simulink model "BMS4Cell"  (R2026a)
settings: Solver=daessc  StopTime=P.StopTime  MaxStep=10  RelTol=1e-4
InitFcn:
  | addpath(fullfile(fileparts(get_param(bdroot, 'FileName')), '..', 'src')); if ~exist('P','var') || ~exist('C','var'), [P, C] = params_4cell('cell'); end
undefined symbols (not defined in the file): C, P
libraries: fl_lib x39, nesl_utility x28, batteryecm_lib x4, ee_lib x4
settings Model: Creator=highdreameater  LastModifiedBy=highdreameater
settings DebuggingCC: AlgebraicLoopMsg=error

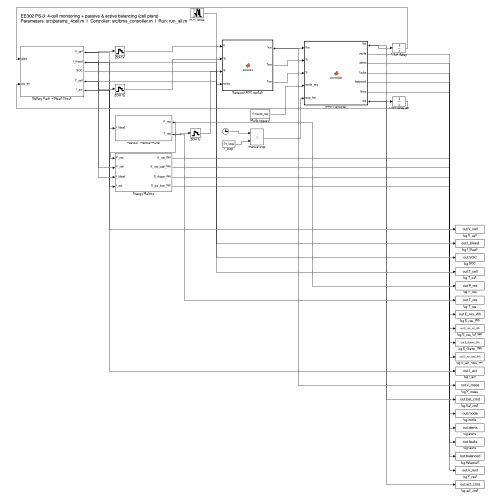
[thumbnail: Simulink's stored preview of the top-level diagram]
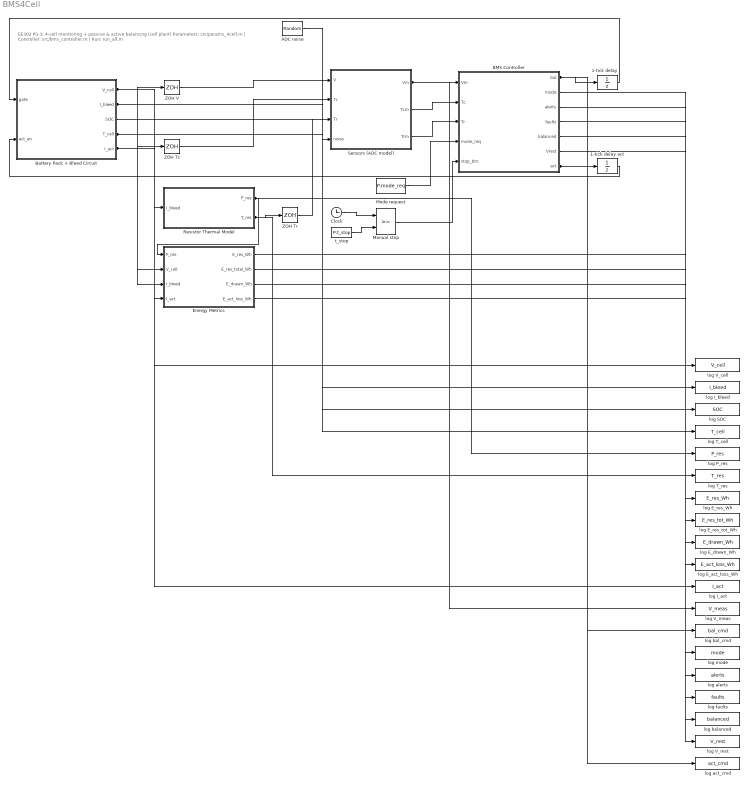
== system BMS4Cell ==
  note: EE302 PS-3: 4-cell monitoring + passive & active balancing (cell plant)
      | Parameters: src/params_4cell.m  |  Controller: src/bms_controller.m  |  Run: run_all.m
  1-tick delay : UnitDelay  InitialCondition=zeros(4,1)  SampleTime=C.Ts
  1-tick delay act : UnitDelay  InitialCondition=zeros(3,1)  SampleTime=C.Ts
  ADC noise : RandomNumber  Mean=zeros(4,1)  Variance=P.noise_V^2*ones(4,1)  Seed=P.seed  SampleTime=C.Ts
  BMS Controller : MATLAB Function  TreatAsAtomicUnit=on
  Battery Pack + Bleed Circuit : Subsystem
  Clock : Clock
  Energy Metrics : Subsystem
  Manual stop : RelationalOperator  OutDataTypeStr=boolean  RndMeth=Simplest  InputSameDT=off
  Mode request : Constant  Value=P.mode_req
  Resistor Thermal Model : Subsystem
  Sensors (ADC model) : MATLAB Function  TreatAsAtomicUnit=on
  ZOH Tc : ZeroOrderHold  SampleTime=C.Ts
  ZOH Tr : ZeroOrderHold  SampleTime=C.Ts
  ZOH V : ZeroOrderHold  SampleTime=C.Ts
  log E_act_loss_Wh : ToWorkspace  VariableName=E_act_loss_Wh  SaveFormat=Timeseries  SampleTime=P.log_dt
  log E_drawn_Wh : ToWorkspace  VariableName=E_drawn_Wh  SaveFormat=Timeseries  SampleTime=P.log_dt
  log E_res_Wh : ToWorkspace  VariableName=E_res_Wh  SaveFormat=Timeseries  SampleTime=P.log_dt
  log E_res_tot_Wh : ToWorkspace  VariableName=E_res_tot_Wh  SaveFormat=Timeseries  SampleTime=P.log_dt
  log I_act : ToWorkspace  VariableName=I_act  SaveFormat=Timeseries  SampleTime=P.log_dt
  log I_bleed : ToWorkspace  VariableName=I_bleed  SaveFormat=Timeseries  SampleTime=P.log_dt
  log P_res : ToWorkspace  VariableName=P_res  SaveFormat=Timeseries  SampleTime=P.log_dt
  log SOC : ToWorkspace  VariableName=SOC  SaveFormat=Timeseries  SampleTime=P.log_dt
  log T_cell : ToWorkspace  VariableName=T_cell  SaveFormat=Timeseries  SampleTime=P.log_dt
  log T_res : ToWorkspace  VariableName=T_res  SaveFormat=Timeseries  SampleTime=P.log_dt
  log V_cell : ToWorkspace  VariableName=V_cell  SaveFormat=Timeseries  SampleTime=P.log_dt
  log V_meas : ToWorkspace  VariableName=V_meas  SaveFormat=Timeseries  SampleTime=C.Ts
  log V_rest : ToWorkspace  VariableName=V_rest  SaveFormat=Timeseries  SampleTime=C.Ts
  log act_cmd : ToWorkspace  VariableName=act_cmd  SaveFormat=Timeseries  SampleTime=C.Ts
  log alerts : ToWorkspace  VariableName=alerts  SaveFormat=Timeseries  SampleTime=C.Ts
  log bal_cmd : ToWorkspace  VariableName=bal_cmd  SaveFormat=Timeseries  SampleTime=C.Ts
  log balanced : ToWorkspace  VariableName=balanced  SaveFormat=Timeseries  SampleTime=C.Ts
  log faults : ToWorkspace  VariableName=faults  SaveFormat=Timeseries  SampleTime=C.Ts
  log mode : ToWorkspace  VariableName=mode  SaveFormat=Timeseries  SampleTime=C.Ts
  t_stop : Constant  Value=P.t_stop
  wires:
  Battery Pack + Bleed Circuit/1(V_cell) -> ZOH V/1, Energy Metrics/2(V_cell), log V_cell/1
  Battery Pack + Bleed Circuit/4(T_cell) -> ZOH Tc/1, log T_cell/1
  Battery Pack + Bleed Circuit/2(I_bleed) -> Resistor Thermal Model/1(I_bleed), Energy Metrics/3(I_bleed), log I_bleed/1
  Resistor Thermal Model/2(T_res) -> ZOH Tr/1, log T_res/1
  Resistor Thermal Model/1(P_res) -> Energy Metrics/1(P_res), log P_res/1
  ZOH V/1 -> Sensors (ADC model)/1(V)
  ZOH Tc/1 -> Sensors (ADC model)/2(Tc)
  ZOH Tr/1 -> Sensors (ADC model)/3(Tr)
  ADC noise/1 -> Sensors (ADC model)/4(noise)
  Sensors (ADC model)/1(Vm) -> BMS Controller/1(Vm), log V_meas/1
  Sensors (ADC model)/2(Tcm) -> BMS Controller/2(Tc)
  Sensors (ADC model)/3(Trm) -> BMS Controller/3(Tr)
  Mode request/1 -> BMS Controller/4(mode_req)
  Clock/1 -> Manual stop/1
  t_stop/1 -> Manual stop/2
  Manual stop/1 -> BMS Controller/5(stop_btn)
  BMS Controller/1(bal) -> 1-tick delay/1, log bal_cmd/1
  1-tick delay/1 -> Battery Pack + Bleed Circuit/1(gate)
  BMS Controller/7(act) -> 1-tick delay act/1, log act_cmd/1
  1-tick delay act/1 -> Battery Pack + Bleed Circuit/2(act_en)
  Battery Pack + Bleed Circuit/5(I_act) -> Energy Metrics/4(I_act), log I_act/1
  Battery Pack + Bleed Circuit/3(SOC) -> log SOC/1
  Energy Metrics/1(E_res_Wh) -> log E_res_Wh/1
  Energy Metrics/2(E_res_total_Wh) -> log E_res_tot_Wh/1
  Energy Metrics/3(E_drawn_Wh) -> log E_drawn_Wh/1
  Energy Metrics/4(E_act_loss_Wh) -> log E_act_loss_Wh/1
  BMS Controller/2(mode) -> log mode/1
  BMS Controller/3(alerts) -> log alerts/1
  BMS Controller/4(faults) -> log faults/1
  BMS Controller/5(balanced) -> log balanced/1
  BMS Controller/6(Vrest) -> log V_rest/1

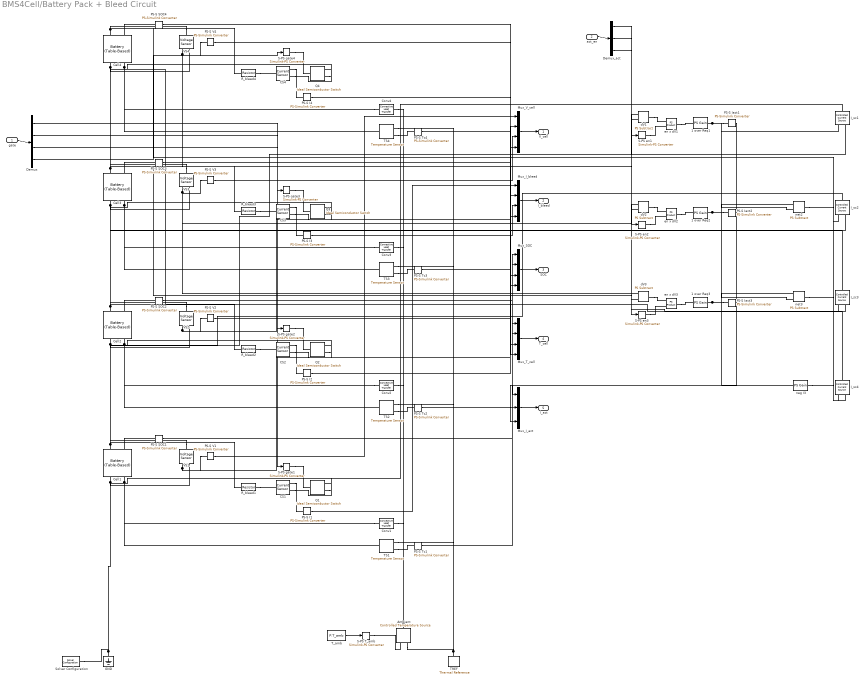
== system BMS4Cell/Battery Pack + Bleed Circuit ==
  gate : Inport
  act_en : Inport  Port=2
  1 over Req1 : fl_lib/Physical Signals/Functions/PS Gain  gain=1/P.R_eq 1/Ohm
  1 over Req2 : fl_lib/Physical Signals/Functions/PS Gain  gain=1/P.R_eq 1/Ohm
  1 over Req3 : fl_lib/Physical Signals/Functions/PS Gain  gain=1/P.R_eq 1/Ohm
  Ambient : fl_lib/Thermal/Thermal Sources/Controlled Temperature Source
  CS{1..4} (4 alike) : fl_lib/Electrical/Electrical Sensors/Current Sensor
  Cell1 : batteryecm_lib/Battery (Table-Based)  SOC_vec=P.SOC_vec  T_dependence=simscape.enum.tablebattery.temperature_dependence.yes  prm_dir=simscape.enum.tablebattery.prm_dir.noCurrentDirectionality  T_vec=P.T_vec K  V0_mat=P.V0_mat V  V0_vec=[3.5057, 3.566, 3.6337, 3.7127, 3.9259, 4.0777, 4.1928] V  V_range=[0, inf] V  R0_mat=P.R0_mat Ohm  R0_vec=[.0085, .0085, .0087, .0082, .0083, .0085, .0085] Ohm  R0_dis_mat=[.0117, .0085, .009; .011, .0085, .009; .0114, .0087, .0092; .0107, .0082, .0088; .0107, .0083, .0091; .0113, .0085, .0089; .0116, .0085, .0089] Ohm  R0_dis_vec=[.0085, .0085, .0087, .0082, .0083, .0085, .0085] Ohm  R0_ch_mat=[.0117, .0085, .009; .011, .0085, .009; .0114, .0087, .0092; .0107, .0082, .0088; .0107, .0083, .0091; .0113, .0085, .0089; .0116, .0085, .0089] Ohm  R0_ch_vec=[.0085, .0085, .0087, .0082, .0083, .0085, .0085] Ohm  AH=P.AH A*hr  prm_leak=simscape.enum.tablebattery.prm_leak.disabled  Rleak_vec=[8000, 7000, 6000] Ohm  Rleak=7e3 Ohm  extrapolation_option=simscape.enum.extrapolation.nearest  SOC_port=simscape.enum.tablebattery.enable.yes  prm_dyn=simscape.enum.tablebattery.prm_dyn.off  R1_mat=[.0109, .0029, .0013; .0069, .0024, .0012; .0047, .0026, .0013; .0034, .0016, .001; .0033, .0023, .0014; .0033, .0018, .0011; .0028, .0017, .0011] Ohm  R1_vec=[.0029, .0024, .0026, .0016, .0023, .0018, .0017] Ohm  tau1_mat=[20, 36, 39; 31, 45, 39; 109, 105, 61; 36, 29, 26; 59, 77, 67; 40, 33, 29; 25, 39, 33] s  tau1_vec=[36, 45, 105, 29, 77, 33, 39] s  R2_mat=[.0109, .0029, .0013; .0069, .0024, .0012; .0047, .0026, .0013; .0034, .0016, .001; .0033, .0023, .0014; .0033, .0018, .0011; .0028, .0017, .0011] Ohm  R2_vec=[.0029, .0024, .0026, .0016, .0023, .0018, .0017] Ohm  tau2_mat=[20, 36, 39; 31, 45, 39; 109, 105, 61; 36, 29, 26; 59, 77, 67; 40, 33, 29; 25, 39, 33] s  tau2_vec=[36, 45, 105, 29, 77, 33, 39] s  R3_mat=[.0109, .0029, .0013; .0069, .0024, .0012; .0047, .0026, .0013; .0034, .0016, .001; .0033, .0023, .0014; .0033, .0018, .0011; .0028, .0017, .0011] Ohm  R3_vec=[.0029, .0024, .0026, .0016, .0023, .0018, .0017] Ohm  tau3_mat=[20, 36, 39; 31, 45, 39; 109, 105, 61; 36, 29, 26; 59, 77, 67; 40, 33, 29; 25, 39, 33] s  tau3_vec=[36, 45, 105, 29, 77, 33, 39] s  R4_mat=[.0109, .0029, .0013; .0069, .0024, .0012; .0047, .0026, .0013; .0034, .0016, .001; .0033, .0023, .0014; .0033, .0018, .0011; .0028, .0017, .0011] Ohm  R4_vec=[.0029, .0024, .0026, .0016, .0023, .0018, .0017] Ohm  tau4_mat=[20, 36, 39; 31, 45, 39; 109, 105, 61; 36, 29, 26; 59, 77, 67; 40, 33, 29; 25, 39, 33] s  tau4_vec=[36, 45, 105, 29, 77, 33, 39] s  R5_mat=[.0109, .0029, .0013; .0069, .0024, .0012; .0047, .0026, .0013; .0034, .0016, .001; .0033, .0023, .0014; .0033, .0018, .0011; .0028, .0017, .0011] Ohm  R5_vec=[.0029, .0024, .0026, .0016, .0023, .0018, .0017] Ohm  tau5_mat=[20, 36, 39; 31, 45, 39; 109, 105, 61; 36, 29, 26; 59, 77, 67; 40, 33, 29; 25, 39, 33] s  tau5_vec=[36, 45, 105, 29, 77, 33, 39] s  prm_fade=simscape.enum.tablebattery.prm_fade.disabled  N0=100  dV0=0  dR0=0  dAH=0  dRleak=0  dR1=0  dR2=0  dR3=0  dR4=0  dR5=0  N0vec=[0, 100, 200, 300]  Tfadevec=[298.15, 323.15] K  dV0vec=[0, 0, 0, 0]  dR0vec=[0, 0, 0, 0]  dAHvec=[0, 0, 0, 0]  dRleakvec=[0, 0, 0, 0]  dR1vec=[0, 0, 0, 0]  dR2vec=[0, 0, 0, 0]  dR3vec=[0, 0, 0, 0]  dR4vec=[0, 0, 0, 0]  dR5vec=[0, 0, 0, 0]  dV0mat=[0, 0; 0, 0; 0, 0; 0, 0]  dR0mat=[0, 0; 0, 0; 0, 0; 0, 0]  dAHmat=[0, 0; 0, 0; 0, 0; 0, 0]  dRleakmat=[0, 0; 0, 0; 0, 0; 0, 0]  dR1mat=[0, 0; 0, 0; 0, 0; 0, 0]  dR2mat=[0, 0; 0, 0; 0, 0; 0, 0]  dR3mat=[0, 0; 0, 0; 0, 0; 0, 0]  dR4mat=[0, 0; 0, 0; 0, 0; 0, 0]  dR5mat=[0, 0; 0, 0; 0, 0; 0, 0]  prm_age_modeling=simscape.enum.tablebattery.prm_age_modeling.equation  storage_dt_age_vec=[0] d  storage_T_age_vec=[273] K  prm_age_OCV=simscape.enum.tablebattery.prm_age_OCV.OCV  OCV_age=0.9  SOC_age=0.6  prm_age_resistance=simscape.enum.tablebattery.prm_age.disabled  OCV_scaling_age_resistance=2.2134e6  OCV_offset_age_resistance=1.632e6  temp_exp_age_resistance=0.515833569 V  t_exp_age_resistance=0.75  T_age_vec_resistance=[273.15, 298.15, 323.15] K  dt_age_vec_resistance=[0, 90, 180, 270] d  dR0_age_vec=[0, 0, 0]  t_meas_dR0_age=100 d  dR0_age_mat=[0, 0, 0; 0, 0, 0; 0, 0, 0; 0, 0, 0]  prm_age_capacity=simscape.enum.tablebattery.prm_age.disabled  OCV_scaling_age_capacity=1.5097e07  OCV_offset_age_capacity=8.3625e06  temp_exp_age_capacity=0.6011 V  t_exp_age_capacity=0.75  T_age_vec_capacity=[273.15, 298.15, 323.15] K  dt_age_vec_capacity=[0, 90, 180, 270] d  dAH_age_vec=[0, 0, 0]  t_meas_dAH_age=100 d  dAH_age_mat=[0, 0, 0; 0, 0, 0; 0, 0, 0; 0, 0, 0]  thermal_port=simscape.enum.thermaleffects.model  temperature=298.15 K  thermal_mass=P.Cth_cell J/K  i_specify=off  i_priority=None  i=0 A  i_nominal_specify=off  i_nominal_value=1  i_nominal_unit=A  v_specify=off  v_priority=None  v=0 V  v_nominal_specify=off  v_nominal_value=1  v_nominal_unit=V  stateOfCharge_specify=on  stateOfCharge_priority=High  stateOfCharge=P.SOC0(1)  stateOfCharge_nominal_specify=off  stateOfCharge_nominal_value=1  stateOfCharge_nominal_unit=1  num_cycles_specify=off  num_cycles_priority=High  num_cycles=0  num_cycles_nominal_specify=off  num_cycles_nominal_value=1  num_cycles_nominal_unit=1  cell_temperature_specify=on  cell_temperature_priority=High  cell_temperature=P.T_amb + 273.15 K  cell_temperature_nominal_specify=off  cell_temperature_nominal_value=1  cell_temperature_nominal_unit=K
  Cell2 : batteryecm_lib/Battery (Table-Based)  SOC_vec=P.SOC_vec  T_dependence=simscape.enum.tablebattery.temperature_dependence.yes  prm_dir=simscape.enum.tablebattery.prm_dir.noCurrentDirectionality  T_vec=P.T_vec K  V0_mat=P.V0_mat V  V0_vec=[3.5057, 3.566, 3.6337, 3.7127, 3.9259, 4.0777, 4.1928] V  V_range=[0, inf] V  R0_mat=P.R0_mat Ohm  R0_vec=[.0085, .0085, .0087, .0082, .0083, .0085, .0085] Ohm  R0_dis_mat=[.0117, .0085, .009; .011, .0085, .009; .0114, .0087, .0092; .0107, .0082, .0088; .0107, .0083, .0091; .0113, .0085, .0089; .0116, .0085, .0089] Ohm  R0_dis_vec=[.0085, .0085, .0087, .0082, .0083, .0085, .0085] Ohm  R0_ch_mat=[.0117, .0085, .009; .011, .0085, .009; .0114, .0087, .0092; .0107, .0082, .0088; .0107, .0083, .0091; .0113, .0085, .0089; .0116, .0085, .0089] Ohm  R0_ch_vec=[.0085, .0085, .0087, .0082, .0083, .0085, .0085] Ohm  AH=P.AH A*hr  prm_leak=simscape.enum.tablebattery.prm_leak.disabled  Rleak_vec=[8000, 7000, 6000] Ohm  Rleak=7e3 Ohm  extrapolation_option=simscape.enum.extrapolation.nearest  SOC_port=simscape.enum.tablebattery.enable.yes  prm_dyn=simscape.enum.tablebattery.prm_dyn.off  R1_mat=[.0109, .0029, .0013; .0069, .0024, .0012; .0047, .0026, .0013; .0034, .0016, .001; .0033, .0023, .0014; .0033, .0018, .0011; .0028, .0017, .0011] Ohm  R1_vec=[.0029, .0024, .0026, .0016, .0023, .0018, .0017] Ohm  tau1_mat=[20, 36, 39; 31, 45, 39; 109, 105, 61; 36, 29, 26; 59, 77, 67; 40, 33, 29; 25, 39, 33] s  tau1_vec=[36, 45, 105, 29, 77, 33, 39] s  R2_mat=[.0109, .0029, .0013; .0069, .0024, .0012; .0047, .0026, .0013; .0034, .0016, .001; .0033, .0023, .0014; .0033, .0018, .0011; .0028, .0017, .0011] Ohm  R2_vec=[.0029, .0024, .0026, .0016, .0023, .0018, .0017] Ohm  tau2_mat=[20, 36, 39; 31, 45, 39; 109, 105, 61; 36, 29, 26; 59, 77, 67; 40, 33, 29; 25, 39, 33] s  tau2_vec=[36, 45, 105, 29, 77, 33, 39] s  R3_mat=[.0109, .0029, .0013; .0069, .0024, .0012; .0047, .0026, .0013; .0034, .0016, .001; .0033, .0023, .0014; .0033, .0018, .0011; .0028, .0017, .0011] Ohm  R3_vec=[.0029, .0024, .0026, .0016, .0023, .0018, .0017] Ohm  tau3_mat=[20, 36, 39; 31, 45, 39; 109, 105, 61; 36, 29, 26; 59, 77, 67; 40, 33, 29; 25, 39, 33] s  tau3_vec=[36, 45, 105, 29, 77, 33, 39] s  R4_mat=[.0109, .0029, .0013; .0069, .0024, .0012; .0047, .0026, .0013; .0034, .0016, .001; .0033, .0023, .0014; .0033, .0018, .0011; .0028, .0017, .0011] Ohm  R4_vec=[.0029, .0024, .0026, .0016, .0023, .0018, .0017] Ohm  tau4_mat=[20, 36, 39; 31, 45, 39; 109, 105, 61; 36, 29, 26; 59, 77, 67; 40, 33, 29; 25, 39, 33] s  tau4_vec=[36, 45, 105, 29, 77, 33, 39] s  R5_mat=[.0109, .0029, .0013; .0069, .0024, .0012; .0047, .0026, .0013; .0034, .0016, .001; .0033, .0023, .0014; .0033, .0018, .0011; .0028, .0017, .0011] Ohm  R5_vec=[.0029, .0024, .0026, .0016, .0023, .0018, .0017] Ohm  tau5_mat=[20, 36, 39; 31, 45, 39; 109, 105, 61; 36, 29, 26; 59, 77, 67; 40, 33, 29; 25, 39, 33] s  tau5_vec=[36, 45, 105, 29, 77, 33, 39] s  prm_fade=simscape.enum.tablebattery.prm_fade.disabled  N0=100  dV0=0  dR0=0  dAH=0  dRleak=0  dR1=0  dR2=0  dR3=0  dR4=0  dR5=0  N0vec=[0, 100, 200, 300]  Tfadevec=[298.15, 323.15] K  dV0vec=[0, 0, 0, 0]  dR0vec=[0, 0, 0, 0]  dAHvec=[0, 0, 0, 0]  dRleakvec=[0, 0, 0, 0]  dR1vec=[0, 0, 0, 0]  dR2vec=[0, 0, 0, 0]  dR3vec=[0, 0, 0, 0]  dR4vec=[0, 0, 0, 0]  dR5vec=[0, 0, 0, 0]  dV0mat=[0, 0; 0, 0; 0, 0; 0, 0]  dR0mat=[0, 0; 0, 0; 0, 0; 0, 0]  dAHmat=[0, 0; 0, 0; 0, 0; 0, 0]  dRleakmat=[0, 0; 0, 0; 0, 0; 0, 0]  dR1mat=[0, 0; 0, 0; 0, 0; 0, 0]  dR2mat=[0, 0; 0, 0; 0, 0; 0, 0]  dR3mat=[0, 0; 0, 0; 0, 0; 0, 0]  dR4mat=[0, 0; 0, 0; 0, 0; 0, 0]  dR5mat=[0, 0; 0, 0; 0, 0; 0, 0]  prm_age_modeling=simscape.enum.tablebattery.prm_age_modeling.equation  storage_dt_age_vec=[0] d  storage_T_age_vec=[273] K  prm_age_OCV=simscape.enum.tablebattery.prm_age_OCV.OCV  OCV_age=0.9  SOC_age=0.6  prm_age_resistance=simscape.enum.tablebattery.prm_age.disabled  OCV_scaling_age_resistance=2.2134e6  OCV_offset_age_resistance=1.632e6  temp_exp_age_resistance=0.515833569 V  t_exp_age_resistance=0.75  T_age_vec_resistance=[273.15, 298.15, 323.15] K  dt_age_vec_resistance=[0, 90, 180, 270] d  dR0_age_vec=[0, 0, 0]  t_meas_dR0_age=100 d  dR0_age_mat=[0, 0, 0; 0, 0, 0; 0, 0, 0; 0, 0, 0]  prm_age_capacity=simscape.enum.tablebattery.prm_age.disabled  OCV_scaling_age_capacity=1.5097e07  OCV_offset_age_capacity=8.3625e06  temp_exp_age_capacity=0.6011 V  t_exp_age_capacity=0.75  T_age_vec_capacity=[273.15, 298.15, 323.15] K  dt_age_vec_capacity=[0, 90, 180, 270] d  dAH_age_vec=[0, 0, 0]  t_meas_dAH_age=100 d  dAH_age_mat=[0, 0, 0; 0, 0, 0; 0, 0, 0; 0, 0, 0]  thermal_port=simscape.enum.thermaleffects.model  temperature=298.15 K  thermal_mass=P.Cth_cell J/K  i_specify=off  i_priority=None  i=0 A  i_nominal_specify=off  i_nominal_value=1  i_nominal_unit=A  v_specify=off  v_priority=None  v=0 V  v_nominal_specify=off  v_nominal_value=1  v_nominal_unit=V  stateOfCharge_specify=on  stateOfCharge_priority=High  stateOfCharge=P.SOC0(2)  stateOfCharge_nominal_specify=off  stateOfCharge_nominal_value=1  stateOfCharge_nominal_unit=1  num_cycles_specify=off  num_cycles_priority=High  num_cycles=0  num_cycles_nominal_specify=off  num_cycles_nominal_value=1  num_cycles_nominal_unit=1  cell_temperature_specify=on  cell_temperature_priority=High  cell_temperature=P.T_amb + 273.15 K  cell_temperature_nominal_specify=off  cell_temperature_nominal_value=1  cell_temperature_nominal_unit=K
  Cell3 : batteryecm_lib/Battery (Table-Based)  SOC_vec=P.SOC_vec  T_dependence=simscape.enum.tablebattery.temperature_dependence.yes  prm_dir=simscape.enum.tablebattery.prm_dir.noCurrentDirectionality  T_vec=P.T_vec K  V0_mat=P.V0_mat V  V0_vec=[3.5057, 3.566, 3.6337, 3.7127, 3.9259, 4.0777, 4.1928] V  V_range=[0, inf] V  R0_mat=P.R0_mat Ohm  R0_vec=[.0085, .0085, .0087, .0082, .0083, .0085, .0085] Ohm  R0_dis_mat=[.0117, .0085, .009; .011, .0085, .009; .0114, .0087, .0092; .0107, .0082, .0088; .0107, .0083, .0091; .0113, .0085, .0089; .0116, .0085, .0089] Ohm  R0_dis_vec=[.0085, .0085, .0087, .0082, .0083, .0085, .0085] Ohm  R0_ch_mat=[.0117, .0085, .009; .011, .0085, .009; .0114, .0087, .0092; .0107, .0082, .0088; .0107, .0083, .0091; .0113, .0085, .0089; .0116, .0085, .0089] Ohm  R0_ch_vec=[.0085, .0085, .0087, .0082, .0083, .0085, .0085] Ohm  AH=P.AH A*hr  prm_leak=simscape.enum.tablebattery.prm_leak.disabled  Rleak_vec=[8000, 7000, 6000] Ohm  Rleak=7e3 Ohm  extrapolation_option=simscape.enum.extrapolation.nearest  SOC_port=simscape.enum.tablebattery.enable.yes  prm_dyn=simscape.enum.tablebattery.prm_dyn.off  R1_mat=[.0109, .0029, .0013; .0069, .0024, .0012; .0047, .0026, .0013; .0034, .0016, .001; .0033, .0023, .0014; .0033, .0018, .0011; .0028, .0017, .0011] Ohm  R1_vec=[.0029, .0024, .0026, .0016, .0023, .0018, .0017] Ohm  tau1_mat=[20, 36, 39; 31, 45, 39; 109, 105, 61; 36, 29, 26; 59, 77, 67; 40, 33, 29; 25, 39, 33] s  tau1_vec=[36, 45, 105, 29, 77, 33, 39] s  R2_mat=[.0109, .0029, .0013; .0069, .0024, .0012; .0047, .0026, .0013; .0034, .0016, .001; .0033, .0023, .0014; .0033, .0018, .0011; .0028, .0017, .0011] Ohm  R2_vec=[.0029, .0024, .0026, .0016, .0023, .0018, .0017] Ohm  tau2_mat=[20, 36, 39; 31, 45, 39; 109, 105, 61; 36, 29, 26; 59, 77, 67; 40, 33, 29; 25, 39, 33] s  tau2_vec=[36, 45, 105, 29, 77, 33, 39] s  R3_mat=[.0109, .0029, .0013; .0069, .0024, .0012; .0047, .0026, .0013; .0034, .0016, .001; .0033, .0023, .0014; .0033, .0018, .0011; .0028, .0017, .0011] Ohm  R3_vec=[.0029, .0024, .0026, .0016, .0023, .0018, .0017] Ohm  tau3_mat=[20, 36, 39; 31, 45, 39; 109, 105, 61; 36, 29, 26; 59, 77, 67; 40, 33, 29; 25, 39, 33] s  tau3_vec=[36, 45, 105, 29, 77, 33, 39] s  R4_mat=[.0109, .0029, .0013; .0069, .0024, .0012; .0047, .0026, .0013; .0034, .0016, .001; .0033, .0023, .0014; .0033, .0018, .0011; .0028, .0017, .0011] Ohm  R4_vec=[.0029, .0024, .0026, .0016, .0023, .0018, .0017] Ohm  tau4_mat=[20, 36, 39; 31, 45, 39; 109, 105, 61; 36, 29, 26; 59, 77, 67; 40, 33, 29; 25, 39, 33] s  tau4_vec=[36, 45, 105, 29, 77, 33, 39] s  R5_mat=[.0109, .0029, .0013; .0069, .0024, .0012; .0047, .0026, .0013; .0034, .0016, .001; .0033, .0023, .0014; .0033, .0018, .0011; .0028, .0017, .0011] Ohm  R5_vec=[.0029, .0024, .0026, .0016, .0023, .0018, .0017] Ohm  tau5_mat=[20, 36, 39; 31, 45, 39; 109, 105, 61; 36, 29, 26; 59, 77, 67; 40, 33, 29; 25, 39, 33] s  tau5_vec=[36, 45, 105, 29, 77, 33, 39] s  prm_fade=simscape.enum.tablebattery.prm_fade.disabled  N0=100  dV0=0  dR0=0  dAH=0  dRleak=0  dR1=0  dR2=0  dR3=0  dR4=0  dR5=0  N0vec=[0, 100, 200, 300]  Tfadevec=[298.15, 323.15] K  dV0vec=[0, 0, 0, 0]  dR0vec=[0, 0, 0, 0]  dAHvec=[0, 0, 0, 0]  dRleakvec=[0, 0, 0, 0]  dR1vec=[0, 0, 0, 0]  dR2vec=[0, 0, 0, 0]  dR3vec=[0, 0, 0, 0]  dR4vec=[0, 0, 0, 0]  dR5vec=[0, 0, 0, 0]  dV0mat=[0, 0; 0, 0; 0, 0; 0, 0]  dR0mat=[0, 0; 0, 0; 0, 0; 0, 0]  dAHmat=[0, 0; 0, 0; 0, 0; 0, 0]  dRleakmat=[0, 0; 0, 0; 0, 0; 0, 0]  dR1mat=[0, 0; 0, 0; 0, 0; 0, 0]  dR2mat=[0, 0; 0, 0; 0, 0; 0, 0]  dR3mat=[0, 0; 0, 0; 0, 0; 0, 0]  dR4mat=[0, 0; 0, 0; 0, 0; 0, 0]  dR5mat=[0, 0; 0, 0; 0, 0; 0, 0]  prm_age_modeling=simscape.enum.tablebattery.prm_age_modeling.equation  storage_dt_age_vec=[0] d  storage_T_age_vec=[273] K  prm_age_OCV=simscape.enum.tablebattery.prm_age_OCV.OCV  OCV_age=0.9  SOC_age=0.6  prm_age_resistance=simscape.enum.tablebattery.prm_age.disabled  OCV_scaling_age_resistance=2.2134e6  OCV_offset_age_resistance=1.632e6  temp_exp_age_resistance=0.515833569 V  t_exp_age_resistance=0.75  T_age_vec_resistance=[273.15, 298.15, 323.15] K  dt_age_vec_resistance=[0, 90, 180, 270] d  dR0_age_vec=[0, 0, 0]  t_meas_dR0_age=100 d  dR0_age_mat=[0, 0, 0; 0, 0, 0; 0, 0, 0; 0, 0, 0]  prm_age_capacity=simscape.enum.tablebattery.prm_age.disabled  OCV_scaling_age_capacity=1.5097e07  OCV_offset_age_capacity=8.3625e06  temp_exp_age_capacity=0.6011 V  t_exp_age_capacity=0.75  T_age_vec_capacity=[273.15, 298.15, 323.15] K  dt_age_vec_capacity=[0, 90, 180, 270] d  dAH_age_vec=[0, 0, 0]  t_meas_dAH_age=100 d  dAH_age_mat=[0, 0, 0; 0, 0, 0; 0, 0, 0; 0, 0, 0]  thermal_port=simscape.enum.thermaleffects.model  temperature=298.15 K  thermal_mass=P.Cth_cell J/K  i_specify=off  i_priority=None  i=0 A  i_nominal_specify=off  i_nominal_value=1  i_nominal_unit=A  v_specify=off  v_priority=None  v=0 V  v_nominal_specify=off  v_nominal_value=1  v_nominal_unit=V  stateOfCharge_specify=on  stateOfCharge_priority=High  stateOfCharge=P.SOC0(3)  stateOfCharge_nominal_specify=off  stateOfCharge_nominal_value=1  stateOfCharge_nominal_unit=1  num_cycles_specify=off  num_cycles_priority=High  num_cycles=0  num_cycles_nominal_specify=off  num_cycles_nominal_value=1  num_cycles_nominal_unit=1  cell_temperature_specify=on  cell_temperature_priority=High  cell_temperature=P.T_amb + 273.15 K  cell_temperature_nominal_specify=off  cell_temperature_nominal_value=1  cell_temperature_nominal_unit=K
  Cell4 : batteryecm_lib/Battery (Table-Based)  SOC_vec=P.SOC_vec  T_dependence=simscape.enum.tablebattery.temperature_dependence.yes  prm_dir=simscape.enum.tablebattery.prm_dir.noCurrentDirectionality  T_vec=P.T_vec K  V0_mat=P.V0_mat V  V0_vec=[3.5057, 3.566, 3.6337, 3.7127, 3.9259, 4.0777, 4.1928] V  V_range=[0, inf] V  R0_mat=P.R0_mat Ohm  R0_vec=[.0085, .0085, .0087, .0082, .0083, .0085, .0085] Ohm  R0_dis_mat=[.0117, .0085, .009; .011, .0085, .009; .0114, .0087, .0092; .0107, .0082, .0088; .0107, .0083, .0091; .0113, .0085, .0089; .0116, .0085, .0089] Ohm  R0_dis_vec=[.0085, .0085, .0087, .0082, .0083, .0085, .0085] Ohm  R0_ch_mat=[.0117, .0085, .009; .011, .0085, .009; .0114, .0087, .0092; .0107, .0082, .0088; .0107, .0083, .0091; .0113, .0085, .0089; .0116, .0085, .0089] Ohm  R0_ch_vec=[.0085, .0085, .0087, .0082, .0083, .0085, .0085] Ohm  AH=P.AH A*hr  prm_leak=simscape.enum.tablebattery.prm_leak.disabled  Rleak_vec=[8000, 7000, 6000] Ohm  Rleak=7e3 Ohm  extrapolation_option=simscape.enum.extrapolation.nearest  SOC_port=simscape.enum.tablebattery.enable.yes  prm_dyn=simscape.enum.tablebattery.prm_dyn.off  R1_mat=[.0109, .0029, .0013; .0069, .0024, .0012; .0047, .0026, .0013; .0034, .0016, .001; .0033, .0023, .0014; .0033, .0018, .0011; .0028, .0017, .0011] Ohm  R1_vec=[.0029, .0024, .0026, .0016, .0023, .0018, .0017] Ohm  tau1_mat=[20, 36, 39; 31, 45, 39; 109, 105, 61; 36, 29, 26; 59, 77, 67; 40, 33, 29; 25, 39, 33] s  tau1_vec=[36, 45, 105, 29, 77, 33, 39] s  R2_mat=[.0109, .0029, .0013; .0069, .0024, .0012; .0047, .0026, .0013; .0034, .0016, .001; .0033, .0023, .0014; .0033, .0018, .0011; .0028, .0017, .0011] Ohm  R2_vec=[.0029, .0024, .0026, .0016, .0023, .0018, .0017] Ohm  tau2_mat=[20, 36, 39; 31, 45, 39; 109, 105, 61; 36, 29, 26; 59, 77, 67; 40, 33, 29; 25, 39, 33] s  tau2_vec=[36, 45, 105, 29, 77, 33, 39] s  R3_mat=[.0109, .0029, .0013; .0069, .0024, .0012; .0047, .0026, .0013; .0034, .0016, .001; .0033, .0023, .0014; .0033, .0018, .0011; .0028, .0017, .0011] Ohm  R3_vec=[.0029, .0024, .0026, .0016, .0023, .0018, .0017] Ohm  tau3_mat=[20, 36, 39; 31, 45, 39; 109, 105, 61; 36, 29, 26; 59, 77, 67; 40, 33, 29; 25, 39, 33] s  tau3_vec=[36, 45, 105, 29, 77, 33, 39] s  R4_mat=[.0109, .0029, .0013; .0069, .0024, .0012; .0047, .0026, .0013; .0034, .0016, .001; .0033, .0023, .0014; .0033, .0018, .0011; .0028, .0017, .0011] Ohm  R4_vec=[.0029, .0024, .0026, .0016, .0023, .0018, .0017] Ohm  tau4_mat=[20, 36, 39; 31, 45, 39; 109, 105, 61; 36, 29, 26; 59, 77, 67; 40, 33, 29; 25, 39, 33] s  tau4_vec=[36, 45, 105, 29, 77, 33, 39] s  R5_mat=[.0109, .0029, .0013; .0069, .0024, .0012; .0047, .0026, .0013; .0034, .0016, .001; .0033, .0023, .0014; .0033, .0018, .0011; .0028, .0017, .0011] Ohm  R5_vec=[.0029, .0024, .0026, .0016, .0023, .0018, .0017] Ohm  tau5_mat=[20, 36, 39; 31, 45, 39; 109, 105, 61; 36, 29, 26; 59, 77, 67; 40, 33, 29; 25, 39, 33] s  tau5_vec=[36, 45, 105, 29, 77, 33, 39] s  prm_fade=simscape.enum.tablebattery.prm_fade.disabled  N0=100  dV0=0  dR0=0  dAH=0  dRleak=0  dR1=0  dR2=0  dR3=0  dR4=0  dR5=0  N0vec=[0, 100, 200, 300]  Tfadevec=[298.15, 323.15] K  dV0vec=[0, 0, 0, 0]  dR0vec=[0, 0, 0, 0]  dAHvec=[0, 0, 0, 0]  dRleakvec=[0, 0, 0, 0]  dR1vec=[0, 0, 0, 0]  dR2vec=[0, 0, 0, 0]  dR3vec=[0, 0, 0, 0]  dR4vec=[0, 0, 0, 0]  dR5vec=[0, 0, 0, 0]  dV0mat=[0, 0; 0, 0; 0, 0; 0, 0]  dR0mat=[0, 0; 0, 0; 0, 0; 0, 0]  dAHmat=[0, 0; 0, 0; 0, 0; 0, 0]  dRleakmat=[0, 0; 0, 0; 0, 0; 0, 0]  dR1mat=[0, 0; 0, 0; 0, 0; 0, 0]  dR2mat=[0, 0; 0, 0; 0, 0; 0, 0]  dR3mat=[0, 0; 0, 0; 0, 0; 0, 0]  dR4mat=[0, 0; 0, 0; 0, 0; 0, 0]  dR5mat=[0, 0; 0, 0; 0, 0; 0, 0]  prm_age_modeling=simscape.enum.tablebattery.prm_age_modeling.equation  storage_dt_age_vec=[0] d  storage_T_age_vec=[273] K  prm_age_OCV=simscape.enum.tablebattery.prm_age_OCV.OCV  OCV_age=0.9  SOC_age=0.6  prm_age_resistance=simscape.enum.tablebattery.prm_age.disabled  OCV_scaling_age_resistance=2.2134e6  OCV_offset_age_resistance=1.632e6  temp_exp_age_resistance=0.515833569 V  t_exp_age_resistance=0.75  T_age_vec_resistance=[273.15, 298.15, 323.15] K  dt_age_vec_resistance=[0, 90, 180, 270] d  dR0_age_vec=[0, 0, 0]  t_meas_dR0_age=100 d  dR0_age_mat=[0, 0, 0; 0, 0, 0; 0, 0, 0; 0, 0, 0]  prm_age_capacity=simscape.enum.tablebattery.prm_age.disabled  OCV_scaling_age_capacity=1.5097e07  OCV_offset_age_capacity=8.3625e06  temp_exp_age_capacity=0.6011 V  t_exp_age_capacity=0.75  T_age_vec_capacity=[273.15, 298.15, 323.15] K  dt_age_vec_capacity=[0, 90, 180, 270] d  dAH_age_vec=[0, 0, 0]  t_meas_dAH_age=100 d  dAH_age_mat=[0, 0, 0; 0, 0, 0; 0, 0, 0; 0, 0, 0]  thermal_port=simscape.enum.thermaleffects.model  temperature=298.15 K  thermal_mass=P.Cth_cell J/K  i_specify=off  i_priority=None  i=0 A  i_nominal_specify=off  i_nominal_value=1  i_nominal_unit=A  v_specify=off  v_priority=None  v=0 V  v_nominal_specify=off  v_nominal_value=1  v_nominal_unit=V  stateOfCharge_specify=on  stateOfCharge_priority=High  stateOfCharge=P.SOC0(4)  stateOfCharge_nominal_specify=off  stateOfCharge_nominal_value=1  stateOfCharge_nominal_unit=1  num_cycles_specify=off  num_cycles_priority=High  num_cycles=0  num_cycles_nominal_specify=off  num_cycles_nominal_value=1  num_cycles_nominal_unit=1  cell_temperature_specify=on  cell_temperature_priority=High  cell_temperature=P.T_amb + 273.15 K  cell_temperature_nominal_specify=off  cell_temperature_nominal_value=1  cell_temperature_nominal_unit=K
  Conv{1..4} (4 alike) : fl_lib/Thermal/Thermal Elements/Convective Heat Transfer  thermal_type=foundation.enum.constant_variable.constant  area=P.A_cell m^2  heat_tr_coeff=P.h_conv W/(K*m^2)  min_heat_tr_coeff=1e-3 W/(K*m^2)  T_specify=off  T_priority=None  T=0 K  T_nominal_specify=off  T_nominal_value=1  T_nominal_unit=K  Q_specify=off  Q_priority=None  Q=0 W  Q_nominal_specify=off  Q_nominal_value=1  Q_nominal_unit=W
  Demux : Demux
  Demux_act : Demux  Outputs=3
  GND : fl_lib/Electrical/Electrical Elements/Electrical Reference
  I_sc{1..4} (4 alike) : fl_lib/Electrical/Electrical Sources/Controlled Current Source
  Mux_I_act : Mux  Inputs=3
  Mux_I_bleed : Mux
  Mux_SOC : Mux
  Mux_T_cell : Mux
  Mux_V_cell : Mux
  PS-S I{1..4} (4 alike) : nesl_utility/PS-Simulink Converter  PhysicalDomain=network_engine_domain  SubClassName=ps_output  LeftPortType=input  RightPortType=output  PseudoPeriodic=off  Frequencies=[]  VectorFormat=inherit  Unit=A  AffineConversion=off
  PS-S Iact1 : nesl_utility/PS-Simulink Converter  PhysicalDomain=network_engine_domain  SubClassName=ps_output  LeftPortType=input  RightPortType=output  PseudoPeriodic=off  Frequencies=[]  VectorFormat=inherit  Unit=A  AffineConversion=off
  PS-S Iact2 : nesl_utility/PS-Simulink Converter  PhysicalDomain=network_engine_domain  SubClassName=ps_output  LeftPortType=input  RightPortType=output  PseudoPeriodic=off  Frequencies=[]  VectorFormat=inherit  Unit=A  AffineConversion=off
  PS-S Iact3 : nesl_utility/PS-Simulink Converter  PhysicalDomain=network_engine_domain  SubClassName=ps_output  LeftPortType=input  RightPortType=output  PseudoPeriodic=off  Frequencies=[]  VectorFormat=inherit  Unit=A  AffineConversion=off
  PS-S SOC{1..4} (4 alike) : nesl_utility/PS-Simulink Converter  PhysicalDomain=network_engine_domain  SubClassName=ps_output  LeftPortType=input  RightPortType=output  PseudoPeriodic=off  Frequencies=[]  VectorFormat=inherit  Unit=1  AffineConversion=off
  PS-S Tc{1..4} (4 alike) : nesl_utility/PS-Simulink Converter  PhysicalDomain=network_engine_domain  SubClassName=ps_output  LeftPortType=input  RightPortType=output  PseudoPeriodic=off  Frequencies=[]  VectorFormat=inherit  Unit=degC  AffineConversion=on
  PS-S V{1..4} (4 alike) : nesl_utility/PS-Simulink Converter  PhysicalDomain=network_engine_domain  SubClassName=ps_output  LeftPortType=input  RightPortType=output  PseudoPeriodic=off  Frequencies=[]  VectorFormat=inherit  Unit=V  AffineConversion=off
  Q{1..4} (4 alike) : ee_lib/Semiconductors & Converters/Ideal Semiconductor Switch  port_option=ee.enum.controlport.ps  Ron=P.R_on Ohm  Goff=1e-6 1/Ohm  Vth=0.5 V  diode_param=ee.enum.semiconductors.protectionDiode.external  diode_Vf=0.8 V  diode_Ron=0.001 Ohm  diode_Goff=1e-5 1/Ohm  diode_C=50e-9 F  diode_iRM=-235 A  diode_iF=300 A  diode_idot=-50 A/us  diode_trr_param=ee.enum.converters.diodetrr.trr_factor  diode_trr_factor=3  diode_trr=15 us  diode_Qrr=1500 s*uA
  R_bleed{1..4} (4 alike) : fl_lib/Electrical/Electrical Elements/Resistor  R=P.R_bleed Ohm  i_specify=off  i_priority=None  i=0 A  i_nominal_specify=off  i_nominal_value=1  i_nominal_unit=A  v_specify=off  v_priority=None  v=0 V  v_nominal_specify=off  v_nominal_value=1  v_nominal_unit=V
  S-PS T_amb : nesl_utility/Simulink-PS Converter  PhysicalDomain=network_engine_domain  SubClassName=ps_input  LeftPortType=input  RightPortType=output  PseudoPeriodic=off  Frequencies=[]  NoiseDistribution=none  NoiseParameters=[]  Unit=degC  AffineConversion=on  FilteringAndDerivatives=provide  SimscapeFilterOrder=1  InputFilterTimeConstant=0.001  UdotUserProvided=0
  S-PS en1 : nesl_utility/Simulink-PS Converter  PhysicalDomain=network_engine_domain  SubClassName=ps_input  LeftPortType=input  RightPortType=output  PseudoPeriodic=off  Frequencies=[]  NoiseDistribution=none  NoiseParameters=[]  Unit=1  AffineConversion=off  FilteringAndDerivatives=provide  SimscapeFilterOrder=1  InputFilterTimeConstant=0.001  UdotUserProvided=0
  S-PS en2 : nesl_utility/Simulink-PS Converter  PhysicalDomain=network_engine_domain  SubClassName=ps_input  LeftPortType=input  RightPortType=output  PseudoPeriodic=off  Frequencies=[]  NoiseDistribution=none  NoiseParameters=[]  Unit=1  AffineConversion=off  FilteringAndDerivatives=provide  SimscapeFilterOrder=1  InputFilterTimeConstant=0.001  UdotUserProvided=0
  S-PS en3 : nesl_utility/Simulink-PS Converter  PhysicalDomain=network_engine_domain  SubClassName=ps_input  LeftPortType=input  RightPortType=output  PseudoPeriodic=off  Frequencies=[]  NoiseDistribution=none  NoiseParameters=[]  Unit=1  AffineConversion=off  FilteringAndDerivatives=provide  SimscapeFilterOrder=1  InputFilterTimeConstant=0.001  UdotUserProvided=0
  S-PS gate{1..4} (4 alike) : nesl_utility/Simulink-PS Converter  PhysicalDomain=network_engine_domain  SubClassName=ps_input  LeftPortType=input  RightPortType=output  PseudoPeriodic=off  Frequencies=[]  NoiseDistribution=none  NoiseParameters=[]  Unit=1  AffineConversion=off  FilteringAndDerivatives=provide  SimscapeFilterOrder=1  InputFilterTimeConstant=0.001  UdotUserProvided=0
  Solver Configuration : nesl_utility/Solver Configuration  PhysicalDomain=network_engine_domain  SubClassName=solver  LeftPortType=input  RightPortType=generic  Tones=[]  Harmonics=[]  SimulateNoise=off  Profile=off  UseLocalSampling=off  EnableSwitchedLinearOptims=on  FrequencyDomain=off  UseCCode=off  RelTol=0.001  AbsTol=0.001  MinStep=1e-09  ToWorkspace=off  RevertToSquareIcSolve=off  NumHomotopyIterations=100  PhasorMode=off  PhasorModeNumHarmonics=1  ConsistencySolver=NEWTON_XTOL_AFTER_FTOL  CanonicalOrdering=CANONICAL  OptimizeIntermediates=OPTIMIZED  IndexReductionMethod=DerivativeReplacement  DoDC=off  ResidualTolerance=1e-09  ConsistencyTolSource=GLOBAL  ConsistencyAbsTol=0.001  ConsistencyRelTol=0.001  ConsistencyTolFactor=0.001  UseLocalSolver=off  LocalSolverChoice=NE_BACKWARD_EULER_ADVANCER  ResolveIndetEquations=on  FunctionEvalNumThread=1  LocalSolverSampleTime=0.001  DoFixedCost=off  MaxNonlinIter=3  MaxModeIter=2  ComputeImpulses=off  ImpulseIterations=2  LinearAlgebra=auto  LinearAlgebraNumThread=0  EquationFormulation=NE_TIME_EF  DelaysMemoryBudget=1024  AutomaticFiltering=on  FilteringTimeConstant=0.001  PartitionStorageMethod=AS_NEEDED  PartitionMemoryBudget=1024  PartitionMethod=ROBUST  MultibodyUseLocalSolver=off  MultibodyLocalSolverChoice=ODE1  MultibodyLocalSolverSampleTime=0.001
  TREF : fl_lib/Thermal/Thermal Elements/Thermal Reference
  TS{1..4} (4 alike) : fl_lib/Thermal/Thermal Sensors/Temperature Sensor  temperature_measure=foundation.enum.MeasurementReference.difference
  T_amb : Constant  Value=P.T_amb
  VS{1..4} (4 alike) : fl_lib/Electrical/Electrical Sensors/Voltage Sensor
  dV1 : fl_lib/Physical Signals/Functions/PS Subtract
  dV2 : fl_lib/Physical Signals/Functions/PS Subtract
  dV3 : fl_lib/Physical Signals/Functions/PS Subtract
  en x dV1 : fl_lib/Physical Signals/Functions/PS Product
  en x dV2 : fl_lib/Physical Signals/Functions/PS Product
  en x dV3 : fl_lib/Physical Signals/Functions/PS Product
  neg I3 : fl_lib/Physical Signals/Functions/PS Gain  gain=-1
  net2 : fl_lib/Physical Signals/Functions/PS Subtract
  net3 : fl_lib/Physical Signals/Functions/PS Subtract
  V_cell : Outport
  I_bleed : Outport  Port=2
  SOC : Outport  Port=3
  T_cell : Outport  Port=4
  I_act : Outport  Port=5
  wires:
  gate/1 -> Demux/1
  act_en/1 -> Demux_act/1
  Mux_V_cell/1 -> V_cell/1
  Mux_I_bleed/1 -> I_bleed/1
  Mux_SOC/1 -> SOC/1
  Mux_T_cell/1 -> T_cell/1
  Mux_I_act/1 -> I_act/1
  T_amb/1 -> S-PS T_amb/1
  PS-S V1/1 -> Mux_V_cell/1
  PS-S I1/1 -> Mux_I_bleed/1
  Demux/1 -> S-PS gate1/1
  PS-S SOC1/1 -> Mux_SOC/1
  PS-S Tc1/1 -> Mux_T_cell/1
  PS-S V2/1 -> Mux_V_cell/2
  PS-S I2/1 -> Mux_I_bleed/2
  Demux/2 -> S-PS gate2/1
  PS-S SOC2/1 -> Mux_SOC/2
  PS-S Tc2/1 -> Mux_T_cell/2
  PS-S V3/1 -> Mux_V_cell/3
  PS-S I3/1 -> Mux_I_bleed/3
  Demux/3 -> S-PS gate3/1
  PS-S SOC3/1 -> Mux_SOC/3
  PS-S Tc3/1 -> Mux_T_cell/3
  PS-S V4/1 -> Mux_V_cell/4
  PS-S I4/1 -> Mux_I_bleed/4
  Demux/4 -> S-PS gate4/1
  PS-S SOC4/1 -> Mux_SOC/4
  PS-S Tc4/1 -> Mux_T_cell/4
  Demux_act/1 -> S-PS en1/1
  PS-S Iact1/1 -> Mux_I_act/1
  Demux_act/2 -> S-PS en2/1
  PS-S Iact2/1 -> Mux_I_act/2
  Demux_act/3 -> S-PS en3/1
  PS-S Iact3/1 -> Mux_I_act/3
  connections:
  GND/LConn1 -- Solver Configuration/RConn1 -- VS1/RConn2 -- Q1/RConn2 -- Cell1/RConn1 -- I_sc1/LConn1
  S-PS T_amb/RConn1 -- Ambient/RConn1
  Ambient/RConn2 -- TS1/RConn1 -- TS2/RConn1 -- TS3/RConn1 -- TREF/LConn1 -- TS4/RConn1
  VS1/LConn1 -- Cell1/LConn1 -- R_bleed1/LConn1 -- VS2/RConn2 -- Q2/RConn2 -- Cell2/RConn1 -- I_sc2/LConn1 -- I_sc1/RConn2
  PS-S V1/LConn1 -- VS1/RConn1 -- dV1/LConn1
  R_bleed1/RConn1 -- CS1/LConn1
  CS1/RConn2 -- Q1/RConn1
  CS1/RConn1 -- PS-S I1/LConn1
  S-PS gate1/RConn1 -- Q1/LConn1
  Cell1/LConn2 -- PS-S SOC1/LConn1
  Conv1/LConn1 -- Cell1/RConn2 -- TS1/LConn1
  Conv1/RConn1 -- Conv2/RConn1 -- Conv3/RConn1 -- Ambient/LConn1 -- Conv4/RConn1
  TS1/RConn2 -- PS-S Tc1/LConn1
  VS2/LConn1 -- Cell2/LConn1 -- R_bleed2/LConn1 -- VS3/RConn2 -- Q3/RConn2 -- Cell3/RConn1 -- I_sc3/LConn1 -- I_sc2/RConn2
  PS-S V2/LConn1 -- VS2/RConn1 -- dV1/LConn2 -- dV2/LConn1
  R_bleed2/RConn1 -- CS2/LConn1
  CS2/RConn2 -- Q2/RConn1
  CS2/RConn1 -- PS-S I2/LConn1
  S-PS gate2/RConn1 -- Q2/LConn1
  Cell2/LConn2 -- PS-S SOC2/LConn1
  Conv2/LConn1 -- Cell2/RConn2 -- TS2/LConn1
  TS2/RConn2 -- PS-S Tc2/LConn1
  VS3/LConn1 -- Cell3/LConn1 -- R_bleed3/LConn1 -- VS4/RConn2 -- Q4/RConn2 -- Cell4/RConn1 -- I_sc4/LConn1 -- I_sc3/RConn2
  PS-S V3/LConn1 -- VS3/RConn1 -- dV2/LConn2 -- dV3/LConn1
  R_bleed3/RConn1 -- CS3/LConn1
  CS3/RConn2 -- Q3/RConn1
  CS3/RConn1 -- PS-S I3/LConn1
  S-PS gate3/RConn1 -- Q3/LConn1
  Cell3/LConn2 -- PS-S SOC3/LConn1
  Conv3/LConn1 -- Cell3/RConn2 -- TS3/LConn1
  TS3/RConn2 -- PS-S Tc3/LConn1
  VS4/LConn1 -- Cell4/LConn1 -- R_bleed4/LConn1 -- I_sc4/RConn2
  PS-S V4/LConn1 -- VS4/RConn1 -- dV3/LConn2
  R_bleed4/RConn1 -- CS4/LConn1
  CS4/RConn2 -- Q4/RConn1
  CS4/RConn1 -- PS-S I4/LConn1
  S-PS gate4/RConn1 -- Q4/LConn1
  Cell4/LConn2 -- PS-S SOC4/LConn1
  Conv4/LConn1 -- Cell4/RConn2 -- TS4/LConn1
  TS4/RConn2 -- PS-S Tc4/LConn1
  dV1/RConn1 -- en x dV1/LConn1
  S-PS en1/RConn1 -- en x dV1/LConn2
  en x dV1/RConn1 -- 1 over Req1/LConn1
  PS-S Iact1/LConn1 -- 1 over Req1/RConn1 -- I_sc1/RConn1 -- net2/LConn2
  dV2/RConn1 -- en x dV2/LConn1
  S-PS en2/RConn1 -- en x dV2/LConn2
  en x dV2/RConn1 -- 1 over Req2/LConn1
  PS-S Iact2/LConn1 -- 1 over Req2/RConn1 -- net2/LConn1 -- net3/LConn2
  dV3/RConn1 -- en x dV3/LConn1
  S-PS en3/RConn1 -- en x dV3/LConn2
  en x dV3/RConn1 -- 1 over Req3/LConn1
  PS-S Iact3/LConn1 -- 1 over Req3/RConn1 -- net3/LConn1 -- neg I3/LConn1
  net2/RConn1 -- I_sc2/RConn1
  net3/RConn1 -- I_sc3/RConn1
  neg I3/RConn1 -- I_sc4/RConn1

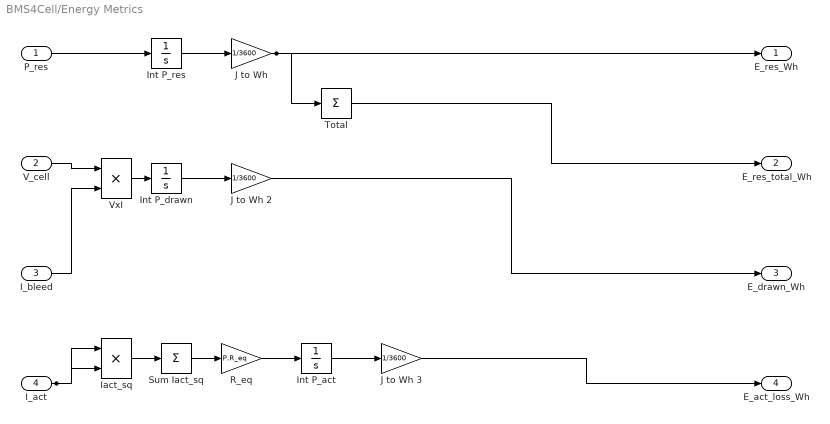
== system BMS4Cell/Energy Metrics ==
  P_res : Inport
  V_cell : Inport  Port=2
  I_bleed : Inport  Port=3
  I_act : Inport  Port=4
  Iact_sq : Product
  Int P_act : Integrator
  Int P_drawn : Integrator
  Int P_res : Integrator
  J to Wh : Gain  Gain=1/3600
  J to Wh 2 : Gain  Gain=1/3600
  J to Wh 3 : Gain  Gain=1/3600
  R_eq : Gain  Gain=P.R_eq
  Sum Iact_sq : Sum  Inputs=+
  Total : Sum  Inputs=+
  VxI : Product
  E_res_Wh : Outport
  E_res_total_Wh : Outport  Port=2
  E_drawn_Wh : Outport  Port=3
  E_act_loss_Wh : Outport  Port=4
  wires:
  P_res/1 -> Int P_res/1
  Int P_res/1 -> J to Wh/1
  J to Wh/1 -> E_res_Wh/1, Total/1
  Total/1 -> E_res_total_Wh/1
  V_cell/1 -> VxI/1
  I_bleed/1 -> VxI/2
  VxI/1 -> Int P_drawn/1
  Int P_drawn/1 -> J to Wh 2/1
  J to Wh 2/1 -> E_drawn_Wh/1
  I_act/1 -> Iact_sq/1, Iact_sq/2
  Iact_sq/1 -> Sum Iact_sq/1
  Sum Iact_sq/1 -> R_eq/1
  R_eq/1 -> Int P_act/1
  Int P_act/1 -> J to Wh 3/1
  J to Wh 3/1 -> E_act_loss_Wh/1

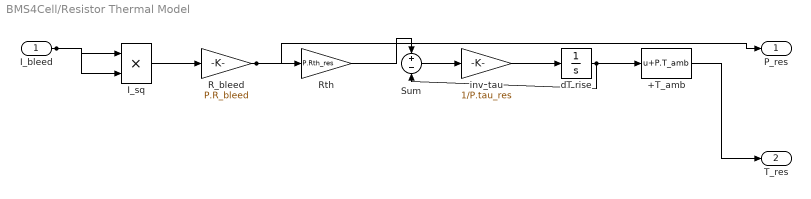
== system BMS4Cell/Resistor Thermal Model ==
  I_bleed : Inport
  +T_amb : Bias  Bias=P.T_amb  SaturateOnIntegerOverflow=off
  I_sq : Product
  R_bleed : Gain  Gain=P.R_bleed
  Rth : Gain  Gain=P.Rth_res
  Sum : Sum  Inputs=+-
  dT rise : Integrator
  inv_tau : Gain  Gain=1/P.tau_res
  P_res : Outport
  T_res : Outport  Port=2
  wires:
  I_bleed/1 -> I_sq/1, I_sq/2
  I_sq/1 -> R_bleed/1
  R_bleed/1 -> Rth/1, P_res/1
  Rth/1 -> Sum/1
  Sum/1 -> inv_tau/1
  inv_tau/1 -> dT rise/1
  dT rise/1 -> Sum/2, +T_amb/1
  +T_amb/1 -> T_res/1

== matlab function BMS4Cell/BMS Controller ==
  data: Vm input; bal output; Tc input; Tr input; mode_req input; stop_btn input; mode output; alerts output; faults output; balanced output; Vrest output; act output; C parameter
function [bal, mode, alerts, faults, balanced, Vrest, act] = controller(Vm, Tc, Tr, mode_req, stop_btn, C)
% Monitoring, passive/active balancing, alerts, faults, manual stop (see bms_controller.m)
[bal, mode, alerts, faults, balanced, Vrest, act] = bms_controller(Vm, Tc, Tr, mode_req, stop_btn, C);

== matlab function BMS4Cell/Sensors (ADC model) ==
  data: V input; Vm output; Tc input; Tr input; noise input; Tcm output; Trm output; C parameter
function [Vm, Tcm, Trm] = sensors(V, Tc, Tr, noise, C)
% Measurement chain: calibration error + noise + ADC quantisation
[Vm, Tcm, Trm] = adc_measure(V, Tc, Tr, noise, C);
